simulink model "SensorlessHFIStartup"  (R2026b)
settings: Solver=ode4  StopTime=hfiStartupTestCfg.Duration  FixedStep=hfiStartupTestCfg.PlantStep
PostLoadFcn:
  | addpath(fullfile(fileparts(get_param(bdroot,'FileName')),'..','build_process'));initialize_hfi_startup(bdroot);
model workspace (MAT data in the model file):
  hfPlantCfg.Rs = 0.5
  hfPlantCfg.Ld = 0.001
  hfPlantCfg.Lq = 0.0015
  hfPlantCfg.Flux = 0.035
  hfPlantCfg.PolePairs = 4
  hfPlantCfg.J = 0.0005
  hfPlantCfg.B = 0.0001
  hfPlantCfg.Id0 = 0
  hfPlantCfg.Iq0 = 0
  hfPlantCfg.Speed0 = 0
  hfPlantCfg.Position0 = 0.175
  hfPlantCfg.SaturationDepth = 0.25
  hfPlantCfg.SaturationCurrent = 1
  hfPlantCfg.CrossInductance = 0
  hfPlantCfg.MechanicalEnabled = 1
  hfPlantCfg.Settings = [0.5; 0.001; 0.0015; 0.035; 4; 0.0005; 0.0001; 0.25; 1; 0; 1]
  hfPlantCfg.InitialState = [0; 0; 0; 0.175]
  hfiCfg.Ts = 5e-05
  hfiCfg.InjectionVoltage = 5
  hfiCfg.Ld = 0.001
  hfiCfg.Lq = 0.0015
  hfiCfg.CrossInductance = 0
  hfiCfg.InitialAxis = 0
  hfiCfg.MaxOmega = 80
  hfiCfg.MinVoltageStep = 1
  hfiCfg.MaxCrossFraction = 0.2
  hfiCfg.MinResponse = 0.01
  hfiCfg.MaxResponse = 0.15
  hfiCfg.MinInjectionScale = 0.1
  hfiCfg.DemodBandwidth = 300
  hfiCfg.DemodFilterEnabled = 1
  hfiCfg.UseMeasuredInverseAverage = 1
  hfiCfg.DemodA = 0.910057240676
  hfiCfg.InverseAverage = 833.333333333
  hfiCfg.CrossPhase = 0
  hfiCfg.InitialTrackerPhase = 0
  hfiCfg.AxisInitialState = [0; 0]
  hfiCfg.DemodSettings = [5e-05; 5; 833.333333333; 0; 1; 0.2; 0.01; 0.15; 0.1; 0.910057240676; 1]
  hfiCfg.TrackSettings = [0; 0; 80]
  hfiStartupTestCfg.Ts = 5e-05
  hfiStartupTestCfg.PlantStep = 2.5e-06
  hfiStartupTestCfg.Duration = 0.3
  hfiStartupTestCfg.InitialElectricalAngle = 0.7
  hfiStartupTestCfg.InitialElectricalSpeed = 0
  hfiStartupTestCfg.SaturationDepth = 0.25
  hfiStartupTestCfg.CrossInductance = 0
  hfiStartupTestCfg.MechanicalEnabled = 1
  hfiStartupTestCfg.Enable = 1
  hfiStartupTestCfg.Reset = 0
  hfiStartupTestCfg.LoadTorque = 0
  hfiStartupTestCfg.MeasurementNoise = 0
  hfiStartupTestCfg.NoiseSeed = 42
  hfiStartupTestCfg.CurrentOffset = [0; 0; 0]
  hfiStartupTestCfg.CurrentResolution = 0
  hfiStartupTestCfg.CurrentRange = 8
  hfiStartupTestCfg.ActuationGain = 1
  hfiStartupTestCfg.ExecutionDelay = 0
  hfiStartupTestCfg.CurrentDelay = 0
  hfiStartupTestCfg.VoltageAlignmentDelay = 0
  hfiStartupTestCfg.PulseNegativeGain = 1
  hfiStartupTestCfg.PulseFaultOffsetA = 0
  hfiStartupTestCfg.QualificationGate = 1
  pllCfg.Ts = 5e-05
  pllCfg.NaturalFrequency = 30
  pllCfg.Damping = 0.707
  pllCfg.Kp = 266.532720731
  pllCfg.Ki = 35530.5758439
  pllCfg.Kaw = 376.991118431
  pllCfg.OmegaMax = 160
  pllCfg.MinMagnitude = 0.01
  pllCfg.LockError = 0.12
  pllCfg.LockSamples = 100
  pllCfg.Theta0 = 0
  pllCfg.Omega0 = 0
  polarityCfg.Ts = 5e-05
  polarityCfg.PulseVoltage = 4
  polarityCfg.PulseTime = 0.001
  polarityCfg.AxisStableTime = 0.005
  polarityCfg.SettleTime = 0.005
  polarityCfg.DecayStableTime = 0.0005
  polarityCfg.AxisTimeout = 0.2
  polarityCfg.StageTimeout = 0.05
  polarityCfg.TotalTimeout = 0.35
  polarityCfg.CurrentDecay = 0.03
  polarityCfg.MaxCurrent = 6
  polarityCfg.MaxAxisSpeed = 2
  polarityCfg.MinPeakDifference = 0.1
  polarityCfg.MinRelativeDifference = 0.03
  polarityCfg.MinPulseDose = 0.001
  polarityCfg.MaxDoseMismatch = 0.05
  polarityCfg.MaxCrossDoseFraction = 0.1
  polarityCfg.MinPulseVoltage = 0.5
  polarityCfg.SpeedFilterTime = 0.005
  polarityCfg.PulseSamples = 20
  polarityCfg.AxisStableSamples = 100
  polarityCfg.SettleSamples = 100
  polarityCfg.DecayStableSamples = 10
  polarityCfg.AxisTimeoutSamples = 4000
  polarityCfg.StageTimeoutSamples = 1000
  polarityCfg.TotalTimeoutSamples = 7000
  polarityCfg.SpeedA = 0.990049833749
  polarityCfg.Settings = [5e-05; 4; 20; 100; 100; 10; 4000; 1000; 7000; 0.03; 6; 2; 0.1; 0.03; 0.001; 0.05; 0.1; 0.5; 0.990049833749]
  polarityCfg.InitialState = [0; 0; 0; 0; 0; 0; 0; 0; 0; 0; 0; 0; 0; 0; 0; 0; 0; 0; 0]
  probeCfg.Ts = 5e-05
  probeCfg.InjectionVoltage = 5
  probeCfg.WarmupSamples = 32
  probeCfg.CaptureSamples = 256
  probeCfg.MinSaliencyRatio = 0.08
  probeCfg.MaxSaliencyRatio = 0.8
  probeCfg.MinInverseInductance = 100
  probeCfg.MaxInverseInductance = 5000
  probeCfg.MaxFitResidual = 0.2
  probeCfg.MaxAsymmetry = 0.1
  probeCfg.MinVoltageRms = 1
  probeCfg.MaxCurrent = 2
  probeCfg.ProbeAxis = 0
  probeCfg.CrossPhase = 0
  probeCfg.Settings = [5e-05; 5; 32; 256; 0.08; 0.8; 100; 5000; 0.2; 0.1; 1; 2; 0; 0]
  probeCfg.InitialState = [0; 0; 0; 0; 0; 0; 0; 0; 0; 0; 0; 0; 0; 0; 0; 0; 0; 0; 0]
  testStim.time = [0 5e-05 0.0001 0.00015 0.0002 0.00025 0.0003 0.00035 0.0004 0.00045 0.0005 0.00055 ... (6001 elements, 6001x1)]
  testStim.signals.values = [0 0 0 0 0 0 0 0 0 0 0 0 ... (42007 elements, 6001x7)]
  testStim.signals.dimensions = 7
libraries: HighFrequencyObserver x3, ClarkePark x2, PMSMHighFrequencyPlant x1
settings Model: Creator=24322  LastModifiedBy=24322

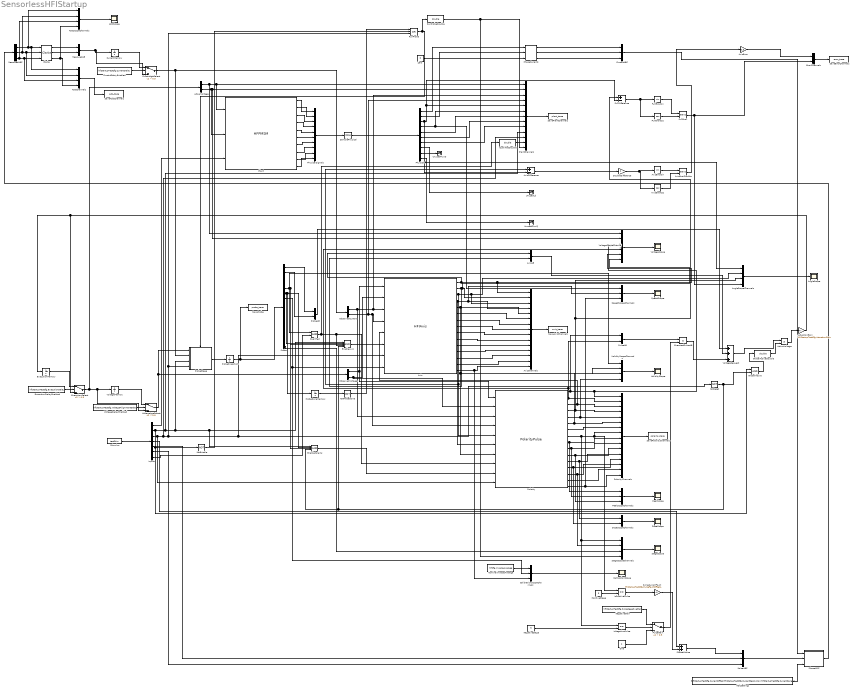
== system SensorlessHFIStartup ==
  ADCChannels : Mux
  ADCScope : Scope
  ADCScopeChannels : Mux
  ADCSettings : Constant  Value=[hfiStartupTestCfg.CurrentOffset;hfiStartupTestCfg.CurrentResolution;hfiStartupTestCfg.CurrentRange]
  ActiveVoltage : Product  Inputs=**
  ActualVoltage : Demux  Outputs=2
  ActuationGain : Gain  Gain=hfiStartupTestCfg.ActuationGain
  AngleScope : Scope
  AngleScopeChannels : Mux
  Axis : HighFrequencyObserver/HFIAxis  cfg=hfiCfg  trackerCfg=pllCfg
  AxisAB : Mux  Inputs=2
  AxisChannels : Mux  Inputs=15
  AxisDifference : Sum  Inputs=+-
  AxisError : Gain  Gain=0.5
  AxisErrorCos : Trigonometry  Operator=cos
  AxisErrorDouble : Trigonometry  Operator=atan2
  AxisErrorSin : Trigonometry
  CalibrationScope : Scope
  CalibrationScopeChannels : Mux  Inputs=3
  Clarke : ClarkePark/Clarke  SystemSampleTime=-1  VariantActivationTime=update diagram  EmptyChoice=off  PassThrough=off  PassThroughVariantControl=(default)  EmptyChoiceVariantControl=(default)  AllowFlexibleInterface=on  Latency=0  AutoFrameSizeCalculation=off
  CurrentABC : Mux  Inputs=3
  CurrentAgeSelect : Switch  Criteria=u2 > Threshold  Threshold=0.5  SaturateOnIntegerOverflow=off  InputSameDT=off
  CurrentDelayEnabled : Constant  Value=hfiStartupTestCfg.CurrentDelay
  CurrentMemory : UnitDelay  InitialCondition=zeros(2,1)  SampleTime=hfiCfg.Ts
  DoseScope : Scope
  DoseScopeChannels : Mux  Inputs=2
  DoubleDifference : Gain  Gain=2
  EnableAxis : Logic  Inputs=5  IconShape=distinctive  AllPortsSameDT=off  OutDataTypeStr=boolean
  EnablePolarity : Logic  Inputs=4  IconShape=distinctive  AllPortsSameDT=off  OutDataTypeStr=boolean
  ErrorChannels : Mux  Inputs=2
  ExecutedPulseAB : Product  Inputs=**
  ExecutionDelayEnabled : Constant  Value=hfiStartupTestCfg.ExecutionDelay
  ExecutionMemory : UnitDelay  InitialCondition=zeros(2,1)  SampleTime=hfiCfg.Ts
  ExecutionSelect : Switch  Criteria=u2 > Threshold  Threshold=0.5  SaturateOnIntegerOverflow=off  InputSameDT=off
  FullDifference : Sum  Inputs=+-
  FullError : Trigonometry  Operator=atan2
  FullErrorCos : Trigonometry  Operator=cos
  FullErrorSin : Trigonometry
  GlobalActive : Logic  AllPortsSameDT=off  OutDataTypeStr=boolean
  GlobalActiveDouble : DataTypeConversion  OutDataTypeStr=double  SaturateOnIntegerOverflow=off  RndMeth=Floor
  Inputs : Demux  Outputs=7
  IsNegativePulse : RelationalOperator  Operator===  OutDataTypeStr=boolean  RndMeth=Simplest  InputSameDT=off
  IsPositivePulse : RelationalOperator  Operator===  OutDataTypeStr=boolean  RndMeth=Simplest  InputSameDT=off
  MeasuredAB : Mux  Inputs=2
  MeasuredABC : Demux  Outputs=3
  NegativeGain : Constant  Value=hfiStartupTestCfg.PulseNegativeGain
  NegativeStage : Constant  Value=5
  NoiseABC : Mux  Inputs=3
  NominalInverseAverage : Constant  Value=hfiCfg.InverseAverage
  NotEnable : Logic  Operator=NOT  IconShape=distinctive  AllPortsSameDT=off  OutDataTypeStr=boolean
  NotProbeDone : Logic  Operator=NOT  IconShape=distinctive  AllPortsSameDT=off  OutDataTypeStr=boolean
  NotReset : Logic  Operator=NOT  IconShape=distinctive  AllPortsSameDT=off  OutDataTypeStr=boolean
  ObservedCurrent : Demux  Outputs=2
  ObservedVoltage : Demux  Outputs=2
  One : Constant
  PeakScope : Scope
  PeakScopeChannels : Mux  Inputs=3
  PhaseADC : MATLAB Function  TreatAsAtomicUnit=on
  PhaseANoise : Sum
  PhaseCurrents : ClarkePark/InverseClarke  SystemSampleTime=-1  VariantActivationTime=update diagram  EmptyChoice=off  PassThrough=off  PassThroughVariantControl=(default)  EmptyChoiceVariantControl=(default)  AllowFlexibleInterface=on  Latency=0  AutoFrameSizeCalculation=off
  Physical : Demux  Outputs=10
  PhysicalSignals : Mux  Inputs=10
  Plant : PMSMHighFrequencyPlant/HFPMSM  cfg=hfPlantCfg
  PlantChannels : Mux  Inputs=13
  Polarity : HighFrequencyObserver/PolarityPulse  cfg=polarityCfg
  PolarityChannels : Mux  Inputs=16
  PositiveStage : Constant  Value=3
  Probe : Demux  Outputs=16
  ProbeAB : Mux  Inputs=2
  ProbeDoneMemory : UnitDelay  SampleTime=hfiCfg.Ts
  ProbeSnapshot : UnitDelay  InitialCondition=zeros(16,1)  SampleTime=hfiCfg.Ts
  ProbeStage : Subsystem
  PulseAB : Mux  Inputs=2
  PulseCurrentFault : Gain  Gain=hfiStartupTestCfg.PulseFaultOffsetA
  PulseGain : Switch  Criteria=u2 > Threshold  Threshold=0.5  SaturateOnIntegerOverflow=off  InputSameDT=off
  Qualified : Logic  IconShape=distinctive  AllPortsSameDT=off  OutDataTypeStr=boolean
  QualifiedDouble : DataTypeConversion  OutDataTypeStr=double  SaturateOnIntegerOverflow=off  RndMeth=Floor
  RunProbe : Logic  Operator=OR  Inputs=3  IconShape=distinctive  AllPortsSameDT=off  OutDataTypeStr=boolean
  RunProbeDouble : DataTypeConversion  OutDataTypeStr=double  SaturateOnIntegerOverflow=off  RndMeth=Floor
  SamplePhysical : ZeroOrderHold  SampleTime=hfiCfg.Ts
  SaveADCChannels : ToWorkspace  VariableName=adc_trace  SaveFormat=Structure With Time  SampleTime=-1
  SaveAxisChannels : ToWorkspace  VariableName=axis_trace  SaveFormat=Structure With Time  SampleTime=-1
  SaveErrorChannels : ToWorkspace  VariableName=error_trace  SaveFormat=Structure With Time  SampleTime=-1
  SavePlantChannels : ToWorkspace  VariableName=plant_trace  SaveFormat=Structure With Time  SampleTime=-1
  SavePolarityChannels : ToWorkspace  VariableName=polarity_trace  SaveFormat=Structure With Time  SampleTime=-1
  SaveProbe : ToWorkspace  VariableName=probe_trace  SaveFormat=Structure With Time  SampleTime=-1
  SpeedScope : Scope
  SpeedScopeChannels : Mux  Inputs=3
  StageScope : Scope
  StageScopeChannels : Mux
  Stimulus : FromWorkspace  VariableName=testStim  SampleTime=hfiCfg.Ts  Interpolate=off  OutputAfterFinalValue=Holding final value
  UnusedFluxD : Terminator
  UnusedFluxQ : Terminator
  UnusedLd : Terminator
  ValidityScope : Scope
  ValidityScopeChannels : Mux
  VoltageAgeSelect : Switch  Criteria=u2 > Threshold  Threshold=0.5  SaturateOnIntegerOverflow=off  InputSameDT=off
  VoltageDelayEnabled : Constant  Value=hfiStartupTestCfg.VoltageAlignmentDelay
  VoltageMemory : UnitDelay  InitialCondition=zeros(2,1)  SampleTime=hfiCfg.Ts
  VoltageRequest : Sum  Inputs=+++
  VoltageScope : Scope
  VoltageScopeChannels : Mux  Inputs=6
  Zero : Constant  Value=0
  wires:
  Stimulus/1 -> Inputs/1
  ProbeDoneMemory/1 -> NotProbeDone/1
  PulseAB/1 -> ExecutedPulseAB/1
  PulseGain/1 -> ExecutedPulseAB/2
  NegativeGain/1 -> PulseGain/1
  IsNegativePulse/1 -> PulseGain/2
  One/1 -> PulseGain/3
  ExecutionMemory/1 -> ExecutionSelect/1
  ExecutionDelayEnabled/1 -> ExecutionSelect/2
  ExecutionSelect/1 -> VoltageMemory/1, VoltageAgeSelect/3, ActualVoltage/1
  VoltageMemory/1 -> VoltageAgeSelect/1
  VoltageDelayEnabled/1 -> VoltageAgeSelect/2
  PhysicalSignals/1 -> SamplePhysical/1
  SamplePhysical/1 -> Physical/1
  CurrentABC/1 -> PhaseADC/1(raw)
  NoiseABC/1 -> PhaseADC/2(noise)
  ADCSettings/1 -> PhaseADC/3(settings)
  PhaseADC/1(measured) -> MeasuredABC/1
  MeasuredAB/1 -> CurrentAgeSelect/3, CurrentMemory/1
  CurrentMemory/1 -> CurrentAgeSelect/1
  CurrentDelayEnabled/1 -> CurrentAgeSelect/2
  Zero/1 -> PhaseCurrents/3
  PhaseANoise/1 -> NoiseABC/1
  IsPositivePulse/1 -> PulseCurrentFault/1
  PulseCurrentFault/1 -> PhaseANoise/2
  NegativeStage/1 -> IsNegativePulse/2
  PositiveStage/1 -> IsPositivePulse/2
  EnableAxis/1 -> Axis/6
  EnablePolarity/1 -> Polarity/9
  AxisDifference/1 -> DoubleDifference/1
  DoubleDifference/1 -> AxisErrorSin/1, AxisErrorCos/1
  AxisErrorSin/1 -> AxisErrorDouble/1
  AxisErrorCos/1 -> AxisErrorDouble/2
  AxisErrorDouble/1 -> AxisError/1
  FullDifference/1 -> FullErrorSin/1, FullErrorCos/1
  FullErrorSin/1 -> FullError/1
  FullErrorCos/1 -> FullError/2
  Inputs/1 -> Plant/3
  Inputs/4 -> PhaseANoise/1
  Inputs/5 -> NoiseABC/2
  Inputs/6 -> NoiseABC/3
  Inputs/7 -> Qualified/2
  Axis/3 -> AxisDifference/1, Polarity/5, AxisChannels/3, AngleScopeChannels/2
  Axis/4 -> AxisChannels/4, SpeedScopeChannels/2, Polarity/6
  Axis/5 -> Polarity/7, ValidityScopeChannels/2, AxisChannels/5
  Polarity/3 -> Axis/5, PolarityChannels/3
  Polarity/8 -> IsNegativePulse/1, StageScopeChannels/1, PolarityChannels/8, IsPositivePulse/1
  Physical/1 -> PhaseCurrents/1
  Physical/2 -> PhaseCurrents/2
  Polarity/4 -> AngleScopeChannels/3, FullDifference/1, PolarityChannels/4
  Physical/8 -> UnusedLd/1
  Physical/9 -> UnusedFluxD/1
  Physical/10 -> UnusedFluxQ/1
  Axis/1 -> AxisChannels/1, VoltageScopeChannels/5, AxisAB/1
  Polarity/1 -> VoltageScopeChannels/3, PolarityChannels/1, PulseAB/1
  ObservedVoltage/1 -> Axis/1, Polarity/1
  Clarke/1 -> MeasuredAB/1
  Axis/2 -> AxisChannels/2, VoltageScopeChannels/6, AxisAB/2
  Polarity/2 -> VoltageScopeChannels/4, PulseAB/2, PolarityChannels/2
  ObservedVoltage/2 -> Axis/2, Polarity/2
  Clarke/2 -> MeasuredAB/2
  PhaseCurrents/1 -> CurrentABC/1
  MeasuredABC/1 -> ADCChannels/1, Clarke/1, ADCScopeChannels/1
  PhaseCurrents/2 -> CurrentABC/2
  MeasuredABC/2 -> ADCChannels/2, Clarke/2, ADCScopeChannels/2
  PhaseCurrents/3 -> CurrentABC/3
  MeasuredABC/3 -> ADCChannels/3, Clarke/3, ADCScopeChannels/3
  Plant/1 -> PhysicalSignals/1
  Plant/2 -> PhysicalSignals/2
  Plant/3 -> PhysicalSignals/3
  Plant/4 -> PhysicalSignals/4
  Plant/5 -> PhysicalSignals/5
  Plant/6 -> PhysicalSignals/6
  Plant/7 -> PhysicalSignals/7
  Plant/8 -> PhysicalSignals/8
  Plant/9 -> PhysicalSignals/9
  Plant/10 -> PhysicalSignals/10
  AxisChannels/1 -> SaveAxisChannels/1
  Axis/6 -> AxisChannels/6
  Axis/7 -> AxisChannels/7
  Axis/8 -> AxisChannels/8
  Axis/9 -> AxisChannels/9
  Axis/10 -> AxisChannels/10
  Axis/11 -> AxisChannels/11
  Axis/12 -> AxisChannels/12
  Axis/13 -> AxisChannels/13
  Axis/14 -> AxisChannels/14
  Axis/15 -> AxisChannels/15, CalibrationScopeChannels/3
  PolarityChannels/1 -> SavePolarityChannels/1
  Polarity/5 -> PolarityChannels/5, ValidityScopeChannels/4
  Polarity/6 -> PolarityChannels/6, ValidityScopeChannels/3
  Polarity/7 -> PolarityChannels/7
  Polarity/9 -> PolarityChannels/9, PeakScopeChannels/1
  Polarity/10 -> PeakScopeChannels/2, PolarityChannels/10
  Polarity/11 -> PeakScopeChannels/3, PolarityChannels/11
  Polarity/12 -> PolarityChannels/12, DoseScopeChannels/1
  Polarity/13 -> DoseScopeChannels/2, PolarityChannels/13
  Polarity/14 -> StageScopeChannels/2, PolarityChannels/14
  Polarity/15 -> PolarityChannels/15
  Polarity/16 -> PolarityChannels/16, SpeedScopeChannels/3
  ErrorChannels/1 -> SaveErrorChannels/1
  AxisError/1 -> ErrorChannels/1
  FullError/1 -> ErrorChannels/2, AngleScopeChannels/4
  ADCChannels/1 -> SaveADCChannels/1
  Clarke/3 -> ADCChannels/4, ADCScopeChannels/4
  AngleScopeChannels/1 -> AngleScope/1
  SpeedScopeChannels/1 -> SpeedScope/1
  ValidityScopeChannels/1 -> ValidityScope/1
  StageScopeChannels/1 -> StageScope/1
  PeakScopeChannels/1 -> PeakScope/1
  DoseScopeChannels/1 -> DoseScope/1
  CalibrationScopeChannels/1 -> CalibrationScope/1
  NominalInverseAverage/1 -> CalibrationScopeChannels/1
  VoltageScopeChannels/1 -> VoltageScope/1
  ADCScopeChannels/1 -> ADCScope/1
  RunProbeDouble/1 -> StageScopeChannels/4, PlantChannels/13
  QualifiedDouble/1 -> PlantChannels/12
  Physical/7 -> PlantChannels/9
  Physical/6 -> PlantChannels/8
  Physical/5 -> PlantChannels/7
  Physical/4 -> SpeedScopeChannels/1, PlantChannels/6
  PlantChannels/1 -> SavePlantChannels/1
  ObservedCurrent/2 -> Polarity/4, Axis/4, PlantChannels/4
  ActualVoltage/2 -> VoltageScopeChannels/2, PlantChannels/2, Plant/2
  ObservedCurrent/1 -> PlantChannels/3, Axis/3, Polarity/3
  ActualVoltage/1 -> Plant/1, PlantChannels/1, VoltageScopeChannels/1
  Physical/3 -> AngleScopeChannels/1, AxisDifference/2, PlantChannels/5, FullDifference/2
  Qualified/1 -> EnableAxis/4, Polarity/8, QualifiedDouble/1
  NotEnable/1 -> RunProbe/2
  NotProbeDone/1 -> RunProbe/1
  ProbeSnapshot/1 -> SaveProbe/1, Probe/1
  RunProbe/1 -> ProbeStage/Enable, RunProbeDouble/1
  Probe/16 -> StageScopeChannels/3
  Probe/2 -> ProbeAB/2
  Probe/1 -> ProbeAB/1
  Probe/7 -> CalibrationScopeChannels/2, Axis/8
  Probe/6 -> EnablePolarity/2, ProbeDoneMemory/1, EnableAxis/2
  Probe/5 -> EnableAxis/3, EnablePolarity/3, Qualified/1, ValidityScopeChannels/1
  CurrentAgeSelect/1 -> ProbeStage/2(current_ab), ObservedCurrent/1
  VoltageAgeSelect/1 -> ProbeStage/1(voltage_ab), ObservedVoltage/1
  ProbeStage/1(snapshot) -> ProbeSnapshot/1
  ActiveVoltage/1 -> ActuationGain/1
  GlobalActiveDouble/1 -> ActiveVoltage/2
  GlobalActive/1 -> GlobalActiveDouble/1
  Inputs/3 -> NotReset/1, Axis/7, RunProbe/3, ProbeStage/4(reset), PlantChannels/11, Polarity/10
  Inputs/2 -> GlobalActive/1, NotEnable/1, EnablePolarity/1, EnableAxis/1, ProbeStage/3(enable), PlantChannels/10
  ActuationGain/1 -> ExecutionMemory/1, ExecutionSelect/3
  VoltageRequest/1 -> ActiveVoltage/1
  ExecutedPulseAB/1 -> VoltageRequest/3
  AxisAB/1 -> VoltageRequest/2
  ProbeAB/1 -> VoltageRequest/1
  NotReset/1 -> EnablePolarity/4, EnableAxis/5, GlobalActive/2

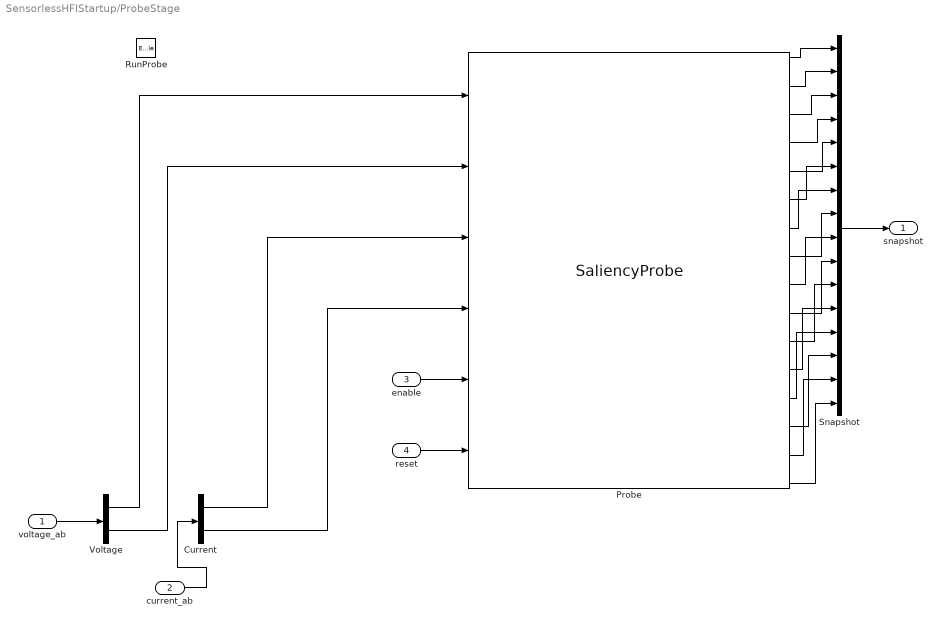
== system SensorlessHFIStartup/ProbeStage ==
  voltage_ab : Inport
  current_ab : Inport  Port=2
  enable : Inport  Port=3
  reset : Inport  Port=4
  RunProbe : EnablePort  StatesWhenEnabling=reset
  Current : Demux  Outputs=2
  Probe : HighFrequencyObserver/SaliencyProbe  cfg=probeCfg
  Snapshot : Mux  Inputs=16
  Voltage : Demux  Outputs=2
  snapshot : Outport  InitialOutput=zeros(16,1)
  wires:
  Probe/16 -> Snapshot/16
  Probe/15 -> Snapshot/15
  Probe/14 -> Snapshot/14
  Probe/13 -> Snapshot/13
  Probe/12 -> Snapshot/12
  Probe/11 -> Snapshot/11
  Probe/10 -> Snapshot/10
  Probe/9 -> Snapshot/9
  Probe/8 -> Snapshot/8
  Probe/7 -> Snapshot/7
  Probe/6 -> Snapshot/6
  Probe/5 -> Snapshot/5
  Probe/4 -> Snapshot/4
  Probe/3 -> Snapshot/3
  Probe/2 -> Snapshot/2
  Probe/1 -> Snapshot/1
  Current/2 -> Probe/4
  Voltage/2 -> Probe/2
  Current/1 -> Probe/3
  Voltage/1 -> Probe/1
  Snapshot/1 -> snapshot/1
  reset/1 -> Probe/6
  enable/1 -> Probe/5
  current_ab/1 -> Current/1
  voltage_ab/1 -> Voltage/1

== matlab function SensorlessHFIStartup/PhaseADC ==
  data: raw input; measured output; noise input; settings input
function measured=hfi_measure_current(raw,noise,settings)
%HFI_MEASURE_CURRENT Three phase ADC fixture: offset, noise, clipping, rounding.
% settings=[offset_a;offset_b;offset_c;resolution_A;range_A].
%#codegen
measured=min(max(raw+noise+settings(1:3),-settings(5)),settings(5));
if settings(4)>0
    measured=round(measured/settings(4))*settings(4);
end
end
